simulink model "final_working_"  (R2021a)
settings: Solver=ode15s  StartTime=0.0  StopTime=3  RelTol=1e-3
libraries: ee_lib x7, nesl_utility x5, fl_lib x4, simulink x1, eeGeneralControl x1, dspstat3 x1, simulink_extras x1, spspowerguiLib x1
settings Model: Creator=Adrija  LastModifiedBy=Adrija
settings SolverCC: ZeroCrossAlgorithm=Adaptive
settings DebuggingCC: IgnoredZcDiagnostic=none

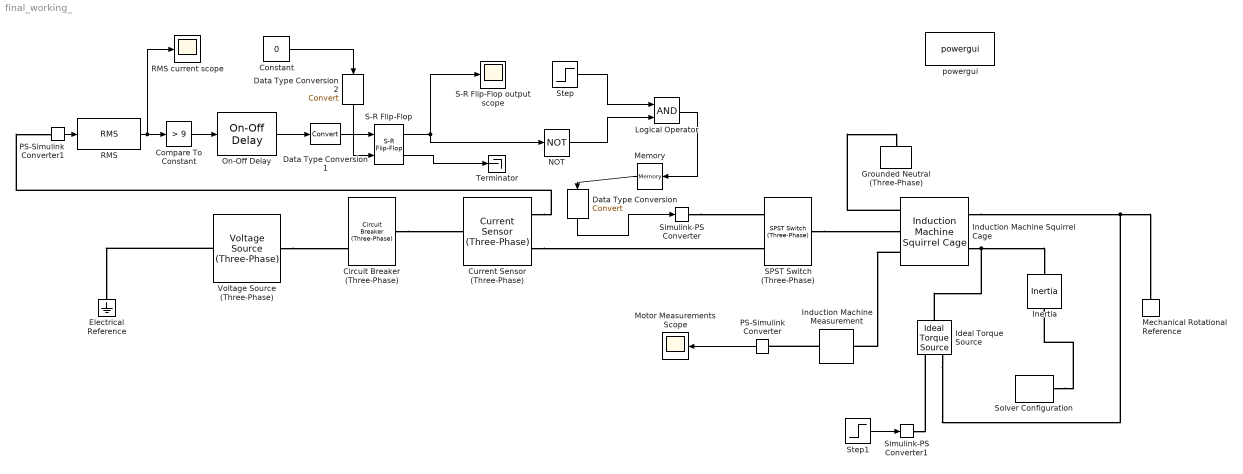
== system final_working_ ==
  Circuit Breaker (Three-Phase) : ee_lib/Switches & Breakers/Circuit Breaker (Three-Phase)  R_closed=0.001 Ohm  G_open=1e-6 1/Ohm  threshold=0.5 V
      settings: SourceProductBaseCode=PS  InternalSimscapePortConfiguration="{\"Bottom\":[],\"Left\":[{\"id\":\"vT\",\"label\":\"vT\",\"type\":\"input\"},{\"id\":\"N1\",\"label\":\"~1\",\"type\":\"foundation.electrical.three_phase\"}],\"Right\":[{\"id\":\"N2\",\"label\":\"~2\",\"type\":\"foundation.electrical.three_phase\"}],\"Top\":[]}"
  Compare To Constant : simulink/Logic and Bit Operations/Compare To Constant  relop=>  const=9  OutDataTypeStr=boolean
  Constant : Constant  Value=0
  Current Sensor (Three-Phase) : ee_lib/Sensors & Transducers/Current Sensor (Three-Phase)
  Data Type Conversion : DataTypeConversion
  Data Type Conversion1 : DataTypeConversion
  Data Type Conversion2 : DataTypeConversion
  Electrical Reference : fl_lib/Electrical/Electrical Elements/Electrical Reference
  Grounded Neutral (Three-Phase) : ee_lib/Connectors & References/Grounded Neutral (Three-Phase)
      settings: SourceProductBaseCode=PS
  Ideal Torque Source : fl_lib/Mechanical/Mechanical Sources/Ideal Torque Source
  Induction Machine Measurement : ee_lib/Electromechanical/Asynchronous/Induction Machine Measurement  output_idx=2
      settings: SourceProductBaseCode=PS  InternalSimscapePortConfiguration="{\"Bottom\":[],\"Left\":[{\"id\":\"pu_input\",\"label\":\"pu\",\"type\":\"input\"}],\"Right\":[{\"id\":\"pu_output\",\"label\":\"o\",\"type\":\"output\"}],\"Top\":[]}"
  Induction Machine Squirrel Cage : ee_lib/Electromechanical/Asynchronous/Induction Machine Squirrel Cage  SRated=15e3 V*A  VRated=220 V  FRated=60 Hz  nPolePairs=1  param_unit=ee.enum.unit.si  squirrel_cage=ee.enum.squirrelcage.Single  zero_sequence=ee.enum.park.zerosequence.exclude  Rs=0.25 Ohm  Xls=0.4 Ohm  pu_Rs=0.0258  pu_Lls=0.0413  Rrd=0.14 Ohm  Xlrd=0.41 Ohm  pu_Rrd=0.0145  pu_Llrd=0.0424  Rrd1=0.28 Ohm  Xlrd1=0.82 Ohm  Rrd2=0.28 Ohm  Xlrd2=0.82 Ohm  pu_Rrd1=0.0290  pu_Llrd1=0.0848  pu_Rrd2=0.0290  pu_Llrd2=0.0848  Xm=17 Ohm  pu_Lm=1.7562  X0=0.4 Ohm  pu_L0=0.0413  saturation_option=ee.enum.saturation.exclude  saturation_i=[0, 4, 9, 18, 25, 34, 50, 68, 95, 120] A  saturation_v=[0, 88, 154, 198, 220, 242, 264, 286, 308, 327] V  pu_saturation_i=[0, .176, .396, .792, 1.1, 1.496, 2.2, 2.992, 4.18, 5.28]  pu_saturation_v=[0, .4, .7, .9, 1, 1.1, 1.2, 1.3, 1.4, 1.4864]  initialization_option=ee.enum.asm.initialization.fluxvariables  connection_option=ee.enum.Connection.delta  angular_position_specify=off  angular_position_priority=None  angular_position=0 deg  angular_position_nominal_specify=off  angular_position_nominal_unit=deg  angular_position_nominal_value=1  pu_psids_specify=off  pu_psids_priority=None  pu_psids=0  pu_psids_nominal_specify=off  pu_psids_nominal_unit=1  pu_psids_nominal_value=1  pu_psiqs_specify=off  pu_psiqs_priority=None  pu_psiqs=0  pu_psiqs_nominal_specify=off  pu_psiqs_nominal_unit=1  pu_psiqs_nominal_value=1  pu_psi0s_specify=off  pu_psi0s_priority=None  pu_psi0s=0  pu_psi0s_nominal_specify=off  pu_psi0s_nominal_unit=1  pu_psi0s_nominal_value=1  pu_psidr_specify=off  pu_psidr_priority=None  pu_psidr=0  pu_psidr_nominal_specify=off  pu_psidr_nominal_unit=1  pu_psidr_nominal_value=1  pu_psiqr_specify=off  pu_psiqr_priority=None  pu_psiqr=0  pu_psiqr_nominal_specify=off  pu_psiqr_nominal_unit=1  pu_psiqr_nominal_value=1  pu_psidr1_specify=off  pu_psidr1_priority=None  pu_psidr1=0  pu_psidr1_nominal_specify=off  pu_psidr1_nominal_unit=1  pu_psidr1_nominal_value=1  pu_psiqr1_specify=off  pu_psiqr1_priority=None  pu_psiqr1=0  pu_psiqr1_nominal_specify=off  pu_psiqr1_nominal_unit=1  pu_psiqr1_nominal_value=1  pu_psidr2_specify=off  pu_psidr2_priority=None  pu_psidr2=0  pu_psidr2_nominal_specify=off  pu_psidr2_nominal_unit=1  pu_psidr2_nominal_value=1  pu_psiqr2_specify=off  pu_psiqr2_priority=None  pu_psiqr2=0  pu_psiqr2_nominal_specify=off  pu_psiqr2_nominal_unit=1  pu_psiqr2_nominal_value=1  psids_specify=off  psids_priority=None  psids=0 Wb  psids_nominal_specify=off  psids_nominal_unit=Wb  psids_nominal_value=1  psiqs_specify=off  psiqs_priority=None  psiqs=0 Wb  psiqs_nominal_specify=off  psiqs_nominal_unit=Wb  psiqs_nominal_value=1  psi0s_specify=off  psi0s_priority=None  psi0s=0 Wb  psi0s_nominal_specify=off  psi0s_nominal_unit=Wb  psi0s_nominal_value=1  psidr_specify=off  psidr_priority=None  psidr=0 Wb  psidr_nominal_specify=off  psidr_nominal_unit=Wb  psidr_nominal_value=1  psiqr_specify=off  psiqr_priority=None  psiqr=0 Wb  psiqr_nominal_specify=off  psiqr_nominal_unit=Wb  psiqr_nominal_value=1  psidr1_specify=off  psidr1_priority=None  psidr1=0 Wb  psidr1_nominal_specify=off  psidr1_nominal_unit=Wb  psidr1_nominal_value=1  psiqr1_specify=off  psiqr1_priority=None  psiqr1=0 Wb  psiqr1_nominal_specify=off  psiqr1_nominal_unit=Wb  psiqr1_nominal_value=1  psidr2_specify=off  psidr2_priority=None  psidr2=0 Wb  psidr2_nominal_specify=off  psidr2_nominal_unit=Wb  psidr2_nominal_value=1  psiqr2_specify=off  psiqr2_priority=None  psiqr2=0 Wb  psiqr2_nominal_specify=off  psiqr2_nominal_unit=Wb  psiqr2_nominal_value=1  slip_specify=off  slip_priority=None  slip=0  slip_nominal_specify=off  slip_nominal_unit=1  slip_nominal_value=1  real_power_generated_specify=off  real_power_generated_priority=None  real_power_generated=0 W  real_power_generated_nominal_specify=off  real_power_generated_nominal_unit=W  real_power_generated_nominal_value=1  mechanical_power_consumed_specify=off  mechanical_power_consumed_priority=None  mechanical_power_consumed=0 W  mechanical_power_consumed_nominal_specify=off  mechanical_power_consumed_nominal_unit=W  mechanical_power_consumed_nominal_value=1
      settings: SourceProductBaseCode=PS  InternalSimscapePortConfiguration="{\"Bottom\":[],\"Left\":[{\"id\":\"R\",\"label\":\"R\",\"type\":\"foundation.mechanical.rotational.rotational\"},{\"id\":\"C\",\"label\":\"C\",\"type\":\"foundation.mechanical.rotational.rotational\"}],\"Right\":[{\"id\":\"pu_output\",\"label\":\"pu\",\"type\":\"output\"},{\"id\":\"N1\",\"label\":\"~1\",\"type\":\"foundation.electrical.three_phase\"},{\"id\":\"N2\",\"label\":\"~2\",\"type\":\"foundation.electrical.three_phase\"}],\"Top\":[]}"
  Inertia : fl_lib/Mechanical/Rotational Elements/Inertia  inertia=0.01 kg*m^2  num_ports=foundation.enum.numPorts2.two  w_specify=off  w_priority=High  w=0 rad/s  w_nominal_specify=off  w_nominal_unit=rad/s  w_nominal_value=1  t_specify=off  t_priority=None  t=0 N*m  t_nominal_specify=off  t_nominal_unit=N*m  t_nominal_value=1
      settings: InternalSimscapePortConfiguration="{\"Bottom\":[],\"Left\":[{\"id\":\"I\",\"label\":\"\",\"type\":\"foundation.mechanical.rotational.rotational\"}],\"Right\":[{\"id\":\"J\",\"label\":\"\",\"type\":\"foundation.mechanical.rotational.rotational\"}],\"Top\":[]}"
  Logical Operator : Logic  AllPortsSameDT=off  OutDataTypeStr=boolean
  Mechanical Rotational Reference : fl_lib/Mechanical/Rotational Elements/Mechanical Rotational Reference
  Memory : Memory
  Motor Measurements Scope : Scope
  NOT : Logic  Operator=NOT  IconShape=distinctive  AllPortsSameDT=off  OutDataTypeStr=boolean
  On-Off Delay : eeGeneralControl/On-Off Delay  LabelModeActiveChoice=Continuous  Td_on=0.45  Td_off=0  IC=0  Ts=0
      settings: SourceProductBaseCode=PS
  PS-Simulink Converter : nesl_utility/PS-Simulink Converter  PhysicalDomain=network_engine_domain  SubClassName=ps_output  LeftPortType=input  RightPortType=output  PseudoPeriodic=off  Frequencies=[]  Unit=inherit  AffineConversion=off
      settings: SourceProductBaseCode=PW,SS
  PS-Simulink Converter1 : nesl_utility/PS-Simulink Converter  PhysicalDomain=network_engine_domain  SubClassName=ps_output  LeftPortType=input  RightPortType=output  PseudoPeriodic=off  Frequencies=[]  Unit=inherit  AffineConversion=off
      settings: SourceProductBaseCode=PW,SS
  RMS : dspstat3/RMS  run=off  directionMode=Each column  dimension=1  InputProcessing=Columns as channels (frame based)  reset_popup=None
  RMS current scope : Scope
  S-R Flip-Flop : simulink_extras/Flip Flops/S-R Flip-Flop  initial_condition=0
  S-R Flip-Flop output scope : Scope
  SPST Switch (Three-Phase) : ee_lib/Switches & Breakers/SPST Switch (Three-Phase)  R_closed=0.001 Ohm  G_open=1e-6 1/Ohm  threshold=0.1 V  i_vT_specify=off  i_vT_priority=None  i_vT=0 A  i_vT_nominal_specify=off  i_vT_nominal_unit=A  i_vT_nominal_value=1  I_specify=off  I_priority=None  I=[ 0 0 0 ] A  I_nominal_specify=off  I_nominal_unit=A  I_nominal_value=1  V_specify=off  V_priority=None  V=[ 0 0 0 ] V  V_nominal_specify=off  V_nominal_unit=V  V_nominal_value=1  i_a_specify=off  i_a_priority=None  i_a=0 A  i_a_nominal_specify=off  i_a_nominal_unit=A  i_a_nominal_value=1  v_a_specify=off  v_a_priority=None  v_a=0 V  v_a_nominal_specify=off  v_a_nominal_unit=V  v_a_nominal_value=1  i_b_specify=off  i_b_priority=None  i_b=0 A  i_b_nominal_specify=off  i_b_nominal_unit=A  i_b_nominal_value=1  v_b_specify=off  v_b_priority=None  v_b=0 V  v_b_nominal_specify=off  v_b_nominal_unit=V  v_b_nominal_value=1  i_c_specify=off  i_c_priority=None  i_c=0 A  i_c_nominal_specify=off  i_c_nominal_unit=A  i_c_nominal_value=1  v_c_specify=off  v_c_priority=None  v_c=0 V  v_c_nominal_specify=off  v_c_nominal_unit=V  v_c_nominal_value=1
      settings: SourceProductBaseCode=PS  InternalSimscapePortConfiguration="{\"Bottom\":[],\"Left\":[{\"id\":\"vT\",\"label\":\"vT\",\"type\":\"input\"},{\"id\":\"N1\",\"label\":\"~1\",\"type\":\"foundation.electrical.three_phase\"}],\"Right\":[{\"id\":\"N2\",\"label\":\"~2\",\"type\":\"foundation.electrical.three_phase\"}],\"Top\":[]}"
  Simulink-PS Converter : nesl_utility/Simulink-PS Converter  PhysicalDomain=network_engine_domain  SubClassName=ps_input  LeftPortType=input  RightPortType=output  PseudoPeriodic=off  Frequencies=[]  NoiseDistribution=none  NoiseParameters=[]  Unit=V  AffineConversion=off  FilteringAndDerivatives=zero  SimscapeFilterOrder=1  InputFilterTimeConstant=0.001  UdotUserProvided=0
      settings: SourceProductBaseCode=PW,SS
  Simulink-PS Converter1 : nesl_utility/Simulink-PS Converter  PhysicalDomain=network_engine_domain  SubClassName=ps_input  LeftPortType=input  RightPortType=output  PseudoPeriodic=off  Frequencies=[]  NoiseDistribution=none  NoiseParameters=[]  Unit=N*m  AffineConversion=off  FilteringAndDerivatives=zero  SimscapeFilterOrder=1  InputFilterTimeConstant=0.001  UdotUserProvided=0
      settings: SourceProductBaseCode=PW,SS
  Solver Configuration : nesl_utility/Solver Configuration  PhysicalDomain=network_engine_domain  SubClassName=solver  LeftPortType=input  RightPortType=generic  Tones=[]  Harmonics=[]  SimulateNoise=off  Profile=off  UseLocalSampling=off  EnableSwitchedLinearOptims=on  FrequencyDomain=off  UseCCode=off  RelTol=0.001  AbsTol=1e-06  MinStep=1e-09  ToWorkspace=off  RevertToSquareIcSolve=off  NumHomotopyIterations=100  PhasorMode=off  PhasorModeNumHarmonics=1  DoDC=off  ResidualTolerance=1e-09  UseLocalSolver=off  LocalSolverChoice=NE_BACKWARD_EULER_ADVANCER  LocalSolverSampleTime=0.001  DoFixedCost=off  MaxNonlinIter=3  MaxModeIter=2  ComputeImpulses=off  ImpulseIterations=2  LinearAlgebra=auto  EquationFormulation=NE_TIME_EF  DelaysMemoryBudget=1024  AutomaticFiltering=on  FilteringTimeConstant=0.001  PartitionStorageMethod=AS_NEEDED  PartitionMemoryBudget=1024  PartitionMethod=ROBUST
      settings: SourceProductBaseCode=PW,SS
  Step : Step  Time=0.1
  Step1 : Step  After=-5
  Terminator : Terminator
  Voltage Source (Three-Phase) : ee_lib/Sources/Voltage Source (Three-Phase)  vline_rms=220 V  shift=0 deg  freq=60 Hz  impedance_option=1  SShortCircuit=1e6 V*A  XR=15  R=0.01 Ohm  L=3.97e-4 H  G_parasitic=0 1/Ohm  harmonic_option=0  harmonic_orders=[5, 7, 11, 13]  harmonic_ratios=[.1, .1, .1, .1]  I_specify=off  I_priority=None  I=[ 0 0 0 ] A  I_nominal_specify=off  I_nominal_unit=A  I_nominal_value=1
      settings: SourceProductBaseCode=PS
  powergui : spspowerguiLib/powergui  Priority=1  SimulationMode=Continuous  SampleTime=50e-6  frequency=60  Iterations=50  frequencyindice=60  Pbase=100e6  ErrMax=1e-4  UnitsV=kV  UnitsW=MW  buscounter=0  FunctionMessages=off  echomessages=off  EnableUseOfTLC=off  CurrentSourceSwitches=off  DisableSnubberDevices=off  DisableRonSwitches=off  DisableVfSwitches=off  DisplayEquations=off  AutomaticDiscreteSolvers=off  SolverType=Tustin/Backward Euler (TBE)  Interpol=off  ExternalGateDelay=off  methode=off  Ts=100  x0status=blocks  SPID=on  SwTol=0  HookPort=off  NonlinearTolerance=1e-4  nMaxIteration=100  ContinueOnMaxIteration=off  RestoreLinks=warning  ResistiveCurrentMeasurement=off  Frange=[0:2:500]  Ylog=off  Xlog=on  ShowGrid=off  save=off  variable=ZData  structure=0  ZoomFFT=off  StartTime=0.0  cycles=1  DisplayStyle=1  fundamental=60  FreqAxis=off  MaxFrequency=1000  frequencyindicesteady=1  RmsSteady=1  display=off
  wires:
  PS-Simulink Converter/1 -> Motor Measurements Scope/1
  PS-Simulink Converter1/1 -> RMS/1
  RMS/1 -> Compare To Constant/1, RMS current scope/1
  Compare To Constant/1 -> On-Off Delay/1
  Step/1 -> Logical Operator/1
  NOT/1 -> Logical Operator/2
  Logical Operator/1 -> Memory/1
  Memory/1 -> Data Type Conversion/1
  On-Off Delay/1 -> Data Type Conversion1/1
  Data Type Conversion1/1 -> S-R Flip-Flop/1
  Constant/1 -> Data Type Conversion2/1
  Data Type Conversion2/1 -> S-R Flip-Flop/2
  S-R Flip-Flop/2 -> Terminator/1
  S-R Flip-Flop/1 -> NOT/1, S-R Flip-Flop output scope/1
  Data Type Conversion/1 -> Simulink-PS Converter/1
  Step1/1 -> Simulink-PS Converter1/1
  connections:
  Induction Machine Measurement/RConn1 -- PS-Simulink Converter/LConn1
  Induction Machine Squirrel Cage/RConn3 -- Grounded Neutral (Three-Phase)/LConn1
  Voltage Source (Three-Phase)/LConn1 -- Electrical Reference/LConn1
  Solver Configuration/RConn1 -- Inertia/RConn1
  Induction Machine Squirrel Cage/LConn2 -- Ideal Torque Source/RConn2 -- Mechanical Rotational Reference/LConn1
  Induction Machine Squirrel Cage/RConn1 -- Induction Machine Measurement/LConn1
  Induction Machine Squirrel Cage/LConn1 -- Ideal Torque Source/LConn1 -- Inertia/LConn1
  Voltage Source (Three-Phase)/RConn1 -- Circuit Breaker (Three-Phase)/LConn2
  Circuit Breaker (Three-Phase)/RConn1 -- Current Sensor (Three-Phase)/LConn1
  Current Sensor (Three-Phase)/RConn2 -- SPST Switch (Three-Phase)/LConn2
  SPST Switch (Three-Phase)/RConn1 -- Induction Machine Squirrel Cage/RConn2
  Current Sensor (Three-Phase)/RConn1 -- PS-Simulink Converter1/LConn1
  Simulink-PS Converter/RConn1 -- SPST Switch (Three-Phase)/LConn1
  Simulink-PS Converter1/RConn1 -- Ideal Torque Source/RConn1
